simulink model "t_drone"  (R2025b)
settings: Solver=ode23t  StartTime=0.0  StopTime=timespot_spl(end)+2  FixedStep=0.01  MaxStep=1e-2  MinStep=1e-13  RelTol=1e-3  AbsTol=1e-3
InitFcn:
  | model = gcs;
  | 
  | configs = evalin('base', get_param([model '/Configurations'], 'Value'));
  | hold_time = evalin('base', get_param([model '/Hold Time'], 'Value'));
  | transistion_time = evalin('base', get_param([model '/Transistion Time'], 'Value'));
  | 
  | if exist('transforms', 'var') == 1
  |     transforms = transforms;
  | else
  |     transforms = false;
  | end
  | 
  | set_drone_configurations
model workspace (MATLAB code in the model file):
  | load('xy_data_membrane.mat');
undefined symbols (not defined in the file): air_rho, battery, drone_leg, filtD_altitude, filtD_attitude, filtD_motor, filtD_pitch, filtD_position, filtD_roll, filtD_yaw, filtM_altitude, filtM_attitude, filtM_pitch, filtM_position, filtM_roll, filtM_yaw, filtSpd_motor, kd_altitude, kd_attitude, kd_motor, kd_pitch, kd_position, kd_roll, kd_yaw, ki_altitude, ki_attitude, ki_motor, ki_pitch, ki_position, ki_roll, ki_yaw, kp_altitude, kp_attitude, kp_motor, kp_pitch, kp_position, kp_roll, kp_yaw, limit_altitude, limit_attitude, limit_motor, limit_pitch, limit_roll, limit_yaw, mass, pkgDensity, pkgSize, planedepth, pos2attitude, propeller, qc_motor, qd_area, qd_drag, spline_data, spline_yaw, timespot_spl, timespots, waypoints, wind_speed, X ... (+2)
libraries: sm_lib x176, nesl_utility x46, fl_lib x37, slpidlib x9, ee_lib x5, simulink_extras x4, sdl_lib x4, simulink x2, batteryecm_lib x1
(part 8 of 8)

== system t_drone/Quadcopter/Wind and Drag/Aerodynamic Drag/drag force Y ==
  area : Inport
  Cd : Inport  Port=2
  v : Inport  Port=3
  Constant : Constant  Value=rho_air/2
  Gain : Gain  Gain=-1
  Product : Product  Inputs=5
  Sign : Signum  ZeroCross=off
  Square : Math  Operator=square
  f : Outport
  wires:
  v/1 -> Sign/1, Square/1
  area/1 -> Product/2
  Sign/1 -> Product/5
  Gain/1 -> f/1
  Cd/1 -> Product/3
  Square/1 -> Product/4
  Product/1 -> Gain/1
  Constant/1 -> Product/1

== system t_drone/Quadcopter/Wind and Drag/Aerodynamic Drag/drag force Z ==
  vz : Inport
  Constant : Constant  Value=rho_air/2
  Constant1 : Constant  Value=area_values.XY
  Constant2 : Constant  Value=drag_coeff.Cd_Z
  Gain : Gain  Gain=-1
  Product : Product  Inputs=5
  Sign : Signum  ZeroCross=off
  Square : Math  Operator=square
  f : Outport
  wires:
  vz/1 -> Sign/1, Square/1
  Gain/1 -> f/1
  Square/1 -> Product/4
  Product/1 -> Gain/1
  Sign/1 -> Product/5
  Constant1/1 -> Product/2
  Constant/1 -> Product/1
  Constant2/1 -> Product/3

== system t_drone/Quadcopter/Wind and Drag/Aerodynamic Drag/drag moment pitch ==
  v : Inport
  Constant : Constant  Value=rho_air/2
  Constant1 : Constant  Value=area_values.Pitch
  Constant2 : Constant  Value=drag_coeff.Pitch
  Gain : Gain  Gain=-1
  Product : Product  Inputs=5
  Sign : Signum  ZeroCross=off
  Square : Math  Operator=square
  f : Outport
  wires:
  Product/1 -> Gain/1
  Constant2/1 -> Product/3
  v/1 -> Sign/1, Square/1
  Constant/1 -> Product/1
  Sign/1 -> Product/5
  Constant1/1 -> Product/2
  Gain/1 -> f/1
  Square/1 -> Product/4

== system t_drone/Quadcopter/Wind and Drag/Aerodynamic Drag/drag moment roll ==
  v : Inport
  Constant : Constant  Value=rho_air/2
  Constant1 : Constant  Value=area_values.Roll
  Constant2 : Constant  Value=drag_coeff.Roll
  Gain : Gain  Gain=-1
  Product : Product  Inputs=5
  Sign : Signum  ZeroCross=off
  Square : Math  Operator=square
  f : Outport
  wires:
  Product/1 -> Gain/1
  v/1 -> Sign/1, Square/1
  Constant/1 -> Product/1
  Constant1/1 -> Product/2
  Constant2/1 -> Product/3
  Square/1 -> Product/4
  Sign/1 -> Product/5
  Gain/1 -> f/1

== system t_drone/Quadcopter/Wind and Drag/Aerodynamic Drag/drag moment yaw ==
  v : Inport
  Constant : Constant  Value=rho_air/2
  Constant1 : Constant  Value=area_values.Yaw
  Constant2 : Constant  Value=drag_coeff.Yaw
  Gain : Gain  Gain=-1
  Product : Product  Inputs=5
  Sign : Signum  ZeroCross=off
  Square : Math  Operator=square
  f : Outport
  wires:
  Constant1/1 -> Product/2
  Sign/1 -> Product/5
  Constant/1 -> Product/1
  v/1 -> Sign/1, Square/1
  Gain/1 -> f/1
  Constant2/1 -> Product/3
  Square/1 -> Product/4
  Product/1 -> Gain/1

== matlab function t_drone/Maneuver Controller/Position Control/Calculate RBI ==
  data: R_BI output; attitude input
function R_BI  = Calculate_RBI(attitude)

phi   = attitude(1);
theta = attitude(2);
psi   = attitude(3);

% obtain the desired state
R_BI = [cos(theta)*cos(psi)                                    cos(theta)*sin(psi)                          -sin(theta);
    -cos(phi)*sin(psi)+sin(phi)*sin(theta)*cos(psi) cos(phi)*cos(psi)+sin(phi)*sin(theta)*sin(psi) sin(phi)*cos(theta);
    sin(phi)*sin(psi)+cos(phi)*sin(theta)*cos(psi) -sin(phi)*cos(psi)+cos(phi)*sin(theta)*sin(psi) cos(phi)*cos(theta)];

end
